simulink model "Robot_Unicycle_Mobile"  (R2024a)
settings: Solver=ode4  StartTime=0.0  StopTime=200  FixedStep=0.01  RelTol=1e-3
libraries: fuzblock x1
settings Model: Creator=scide  LastModifiedBy=scide

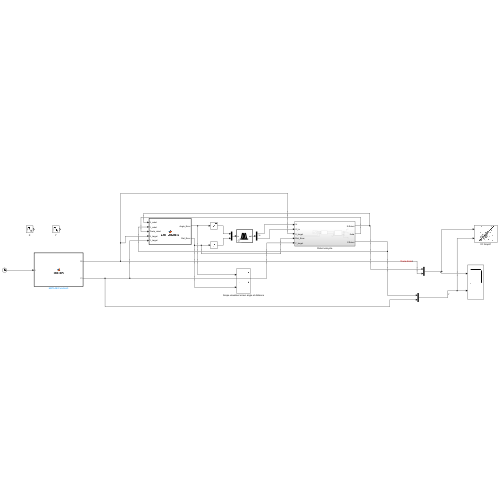
[thumbnail: Simulink's stored preview of the top-level diagram]
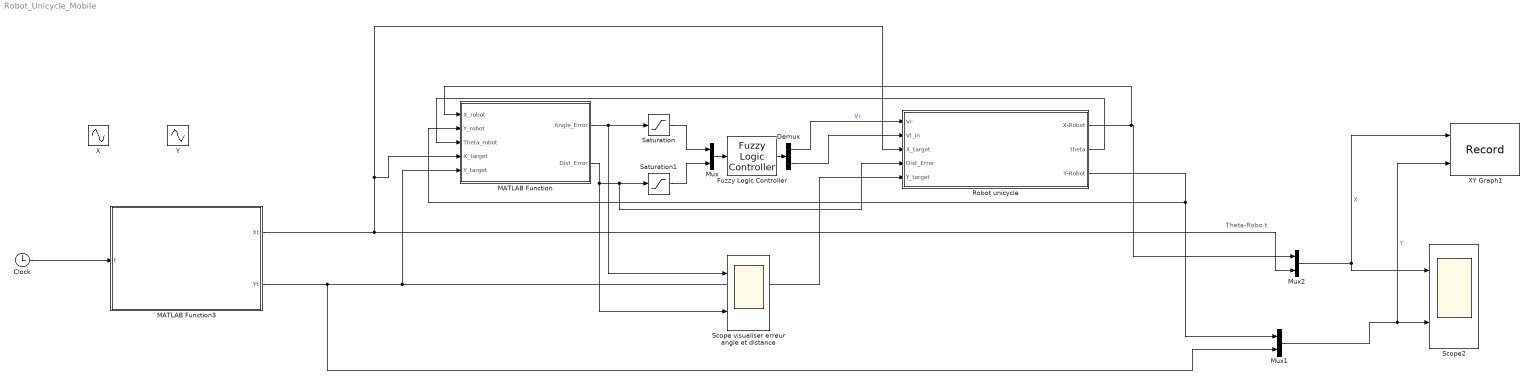
== system Robot_Unicycle_Mobile ==
  note: Theta-Robo t
  Clock : Clock
  Demux : Demux  Outputs=2
  Fuzzy Logic Controller : fuzblock/Fuzzy Logic  Controller  FIS='MobileRobot_3MF.fis'  OutputSampleNumber=101  DataType=double  FuzzifiedInputs=off  RuleFiringStrengths=off  RuleOutputs=off  AggregatedOutputs=off  SimulateUsing=Interpreted execution  OutOfRangeInputValueMessage=warning  NoRuleFiredMessage=warning  EmptyOutputFuzzySetMessage=warning
  MATLAB Function : MATLAB Function  TreatAsAtomicUnit=on
  MATLAB Function3 : MATLAB Function  TreatAsAtomicUnit=on
  Mux : Mux  Inputs=2
  Mux1 : Mux  Inputs=2
  Mux2 : Mux  Inputs=2
  Robot unicycle : Subsystem
  Saturation : Saturate  UpperLimit=1  LowerLimit=-1
  Saturation1 : Saturate  UpperLimit=6.5  LowerLimit=0
  Scope visualiser erreur angle et distance : Scope  NumInputPorts=2
  Scope2 : Scope  NumInputPorts=2
  X : Sin  Amplitude=10  Frequency=0.1  SampleTime=0.01
  XY Graph1 : Record  FileSettingsInternal="{\"entries\":[{\"content\":{\"excelSettings\":{\"content\":{},\"type\":\"Streamout.ExcelSettings\"}},\"type\":\"Streamout.FileSettingStorage\",\"uuid\":\"\"}],\"packageUris\":[\"http:\\/\\/schema.mathworks.com\\/mf0\\/streamout_blocks\\/R2020a\"],\"version\":\"1.0\"}"  Layout=[1 1]  SignalsInternal="{\"entries\":[{\"content\":{\"signals\":[{\"content\":{\"blockPath\":[],\"dimensions\":[2],\"domain\":\"\",\"hasChildren\":true,\"lineColor\":\"#64d413\",\"lineWidth\":2,\"port\":1,\"sid\":[\"\"],\"signalID\":1,\"signalName\":\"X\"},\"type\":\"RecordBlkView.Signal\",\"uuid\":\"\"},{\"content\":{\"blockPath\":[],\"channel\":[1],\"dimensions\":[2],\"domain\":\"\",\"lineColor\":\"#ff13a6\",\"lineWidth\":2,\"parentID\":1,\"plots\":[ 1 ],\"port\":1,\"sid\":[\"\"],\"signalID\":2,\"signalName\":\"X\"},\"type\":\"RecordBlkView.Signal\",\"uuid\":\"\"},{\"content\":{\"blockPath\":[],\"dimensions\":[2],\"domain\":\"\",\"hasChildren\":true,\"lineColor\":\"#fe330a\",\"lineWidth\":2,\"port\":2,\"sid\":[\"\"],\"signalID\":3,\"signalName\":\"Y\"},\"type\":\"RecordBlkView.Signal\",\"uuid\":\"\"},{\"content\":{\"blockPath\":[],\"channel\":[1],\"dimensions\":[2],\"domain\":\"\",\"lineColor\":\"#22b573\",\"lineWidth\":2,\"parentID\":3,\"plots\":[ 1 ],\"port\":2,\"sid\":[\"\"],\"signalID\":4,\"signalName\":\"Y\"},\"type\":\"RecordBlkView.Signal\",\"uuid\":\"\"},{\"content\":{\"blockPath\":[],\"channel\":[2],\"dimensions\":[2],\"domain\":\"\",\"lineColor\":\"#0072bd\",\"lineWidth\":2,\"parentID\":1,\"plots\":[ 1 ],\"port\":1,\"sid\":[\"\"],\"signalID\":5,\"signalName\":\"X\"},\"type\":\"RecordBlkView.Signal\",\"uuid\":\"\"},{\"content\":{\"blockPath\":[],\"channel\":[2],\"dimensions\":[2],\"domain\":\"\",\"lineColor\":\"#d95319\",\"lineWidth\":2,\"parentID\":3,\"plots\":[ 1 ],\"port\":2,\"sid\":[\"\"],\"signalID\":6,\"signalName\":\"Y\"},\"type\":\"RecordBlkView.Signal\",\"uuid\":\"\"}]},\"type\":\"RecordBlkView.InputSignals\",\"uuid\":\"\"}],\"packageUris\":[\"http:\\/\\/schema.mathworks.com\\/mf0\\/streamout_blocks\\/R2020a\"],\"version\":\"1.0\"}"  VisualizationBindings="{\"xyplotplugin\":{\"info\":[{\"series\":[{\"bindingParametersList\":[{\"parameter\":\"X-Axis\",\"signalID\":5,\"signalName\":\"X(2)\"},{\"parameter\":\"Y-Axis\",\"signalID\":6,\"signalName\":\"Y(2)\"},{\"parameter\":\"X-Axis\",\"signalID\":5,\"signalName\":\"X(2)\"},{\"parameter\":\"Y-Axis\",\"signalID\":6,\"signalName\":\"Y(2)\"}],\"seriesID\":0},{\"bindingParametersList\":[{\"parameter\":\"X-Axis\",\"signalID\":2,\"signalName\":\"X(1)\"},{\"parameter\":\"Y-Axis\",\"signalID\":4,\"signalName\":\"Y(1)\"}],\"seriesID\":1}],\"subplotID\":1}]}}"  CompatibilityTag=XY
  Y : Sin  Amplitude=5  Frequency=0.2  SampleTime=0.01
  wires:
  Mux/1 -> Fuzzy Logic Controller/1
  MATLAB Function3/1(Xt) -> MATLAB Function/4(X_target), Robot unicycle/3(X_target), Mux2/2
  MATLAB Function3/2(Yt) -> MATLAB Function/5(Y_target), Robot unicycle/5(Y_target), Mux1/2
  Mux2/1 -> Scope2/1, XY Graph1/1  "X"
  Mux1/1 -> XY Graph1/2, Scope2/2  "Y"
  Clock/1 -> MATLAB Function3/1(t)
  MATLAB Function/1(Angle_Error) -> Scope visualiser erreur angle et distance/1, Saturation/1
  MATLAB Function/2(Dist_Error) -> Scope visualiser erreur angle et distance/2, Robot unicycle/4(Dist_Error), Saturation1/1
  Saturation/1 -> Mux/1
  Saturation1/1 -> Mux/2
  Fuzzy Logic Controller/1 -> Demux/1
  Robot unicycle/3(Y-Robot) -> Mux1/1, MATLAB Function/2(Y_robot)
  Robot unicycle/1(X-Robot) -> MATLAB Function/1(X_robot), Mux2/1
  Demux/1 -> Robot unicycle/1(Vr)  "Vr"
  Demux/2 -> Robot unicycle/2(Vl_in)
  Robot unicycle/2(theta) -> MATLAB Function/3(Theta_robot)

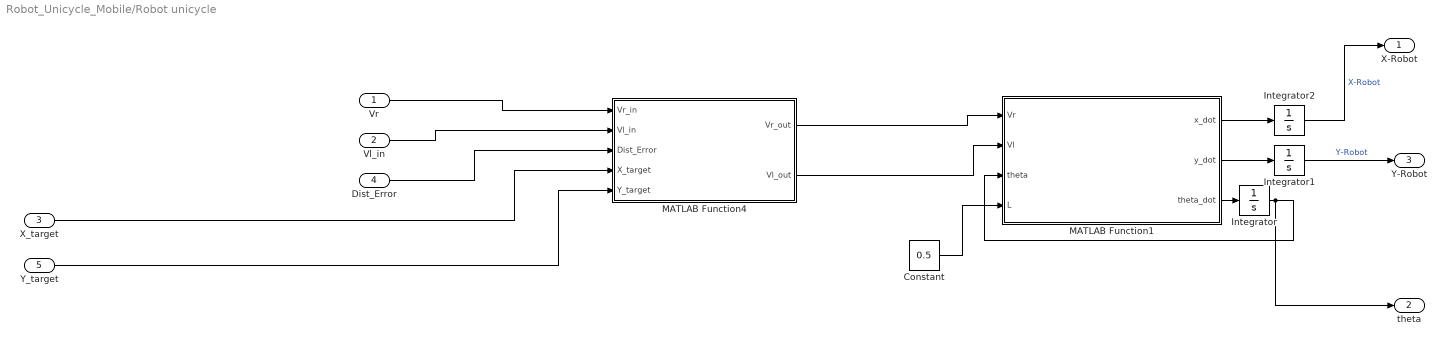
== system Robot_Unicycle_Mobile/Robot unicycle ==
  Vr : Inport
  Vl_in : Inport  Port=2
  X_target : Inport  Port=3
  Dist_Error : Inport  Port=4
  Y_target : Inport  Port=5
  Constant : Constant  Value=0.5
  Integrator : Integrator
  Integrator1 : Integrator
  Integrator2 : Integrator
  MATLAB Function1 : MATLAB Function  TreatAsAtomicUnit=on
  MATLAB Function4 : MATLAB Function  TreatAsAtomicUnit=on
  X-Robot : Outport
  theta : Outport  Port=2
  Y-Robot : Outport  Port=3
  wires:
  MATLAB Function1/1(x_dot) -> Integrator2/1
  Integrator/1 -> theta/1, MATLAB Function1/3(theta)
  Constant/1 -> MATLAB Function1/4(L)
  MATLAB Function4/2(Vl_out) -> MATLAB Function1/2(Vl)
  MATLAB Function1/2(y_dot) -> Integrator1/1
  MATLAB Function4/1(Vr_out) -> MATLAB Function1/1(Vr)
  MATLAB Function1/3(theta_dot) -> Integrator/1
  Integrator2/1 -> X-Robot/1  "X-Robot"
  Integrator1/1 -> Y-Robot/1  "Y-Robot"
  Y_target/1 -> MATLAB Function4/5(Y_target)
  Dist_Error/1 -> MATLAB Function4/3(Dist_Error)
  Vr/1 -> MATLAB Function4/1(Vr_in)
  X_target/1 -> MATLAB Function4/4(X_target)
  Vl_in/1 -> MATLAB Function4/2(Vl_in)

== matlab function Robot_Unicycle_Mobile/Robot unicycle/MATLAB Function1 ==
  data: Vr input; x_dot output; Vl input; theta input; L input; y_dot output; theta_dot output
function [x_dot, y_dot, theta_dot] = Kinematic_Model(Vr, Vl, theta, L)
    
    V = (Vr + Vl) / 2;
    
   
    w = (Vr - Vl) / L;
    
    
    x_dot = V * cos(theta);
    y_dot = V * sin(theta);
    theta_dot = w;
end

== matlab function Robot_Unicycle_Mobile/MATLAB Function ==
  data: X_robot input; Angle_Error output; Y_robot input; Theta_robot input; X_target input; Y_target input; Dist_Error output
function [Angle_Error, Dist_Error] = Error_Calculation(X_robot, Y_robot, Theta_robot, X_target, Y_target)
    % 1. Calcul des différences brutes
    dx = X_target - X_robot;
    dy = Y_target - Y_robot;
    
    % 2. Calcul de la distance
    Dist_Error = sqrt(dx^2 + dy^2);
    
    % 3. Calcul de l'angle
   
    angle_target = atan2(dy, dx);
    e_theta = angle_target - Theta_robot;
    
    % Normalisation entre -pi et pi
    while e_theta > pi
        e_theta = e_theta - 2*pi;
    end
    while e_theta <= -pi
        e_theta = e_theta + 2*pi;
    end
    
   
        Angle_Error = e_theta;
    
    % ---------------------------------------
end

== matlab function Robot_Unicycle_Mobile/MATLAB Function3 ==
  data: t input; Xt output; Yt output
function [Xt, Yt] = Trajectoire(t)
    
    T_fin_trajectoire = 63; 
    
    
    if t < T_fin_trajectoire
        % Paramètres du 8 (Lissajous)
        A = 10;
        omega = 0.1;
        
        Xt = A * sin(omega * t);
        Yt = 5 * sin(2 * omega * t);
        
    % Phase 2 : Parking (Retour à la base)
    else
        
        % On définit une cible fixe.
        Xt = 5;  
        Yt = 5;
    end
end

== matlab function Robot_Unicycle_Mobile/Robot unicycle/MATLAB Function4 ==
  data: Vr_in input; Vr_out output; Vl_in input; Dist_Error input; Vl_out output; X_target input; Y_target input
function [Vr_out, Vl_out] = Gain(Vr_in, Vl_in, Dist_Error, X_target, Y_target)
    
    Dist_Approche = 1.0; % Commence à ralentir à 1m
    Dist_Stop = 0.05;    % S'arrête à 5cm
    
   
    if Dist_Error < Dist_Stop
        Gain = 0; % Freinage total 


    elseif Dist_Error < Dist_Approche
        Gain = (Dist_Error - Dist_Stop) / (Dist_Approche - Dist_Stop);
        Gain = max(Gain, 0.2); 

    else
        Gain = 1; % Pleine puissance
    end
    
    Vr_out = Vr_in * Gain;
    Vl_out = Vl_in * Gain;
end
